simulink model "ECM_1RC_simscape_pulse"  (R2025b)
settings: Solver=ode23t  StartTime=0.0  StopTime=4000  MaxStep=0.1  RelTol=1e-3
libraries: fl_lib x8, nesl_utility x4
settings Model: Creator=klouz  LastModifiedBy=SAT

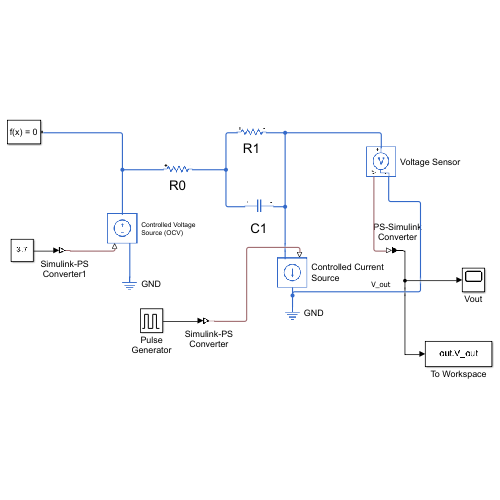
[thumbnail: Simulink's stored preview of the top-level diagram]
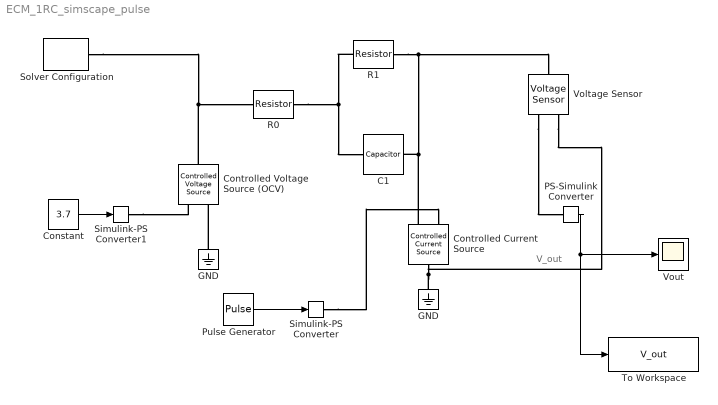
== system ECM_1RC_simscape_pulse ==
  note: V_out
  C1 : fl_lib/Electrical/Electrical Elements/Capacitor  c=1000 F  r=1e-6 Ohm  g=0 1/Ohm  i_specify=off  i_priority=None  i=0 A  i_nominal_specify=off  i_nominal_value=1  i_nominal_unit=A  v_specify=off  v_priority=None  v=0 V  v_nominal_specify=off  v_nominal_value=1  v_nominal_unit=V  vc_specify=off  vc_priority=High  vc=0 V  vc_nominal_specify=off  vc_nominal_value=1  vc_nominal_unit=V
  Constant : Constant  Value=3.7
  Controlled Current Source : fl_lib/Electrical/Electrical Sources/Controlled Current Source
  "Controlled Voltage Source (OCV)  " : fl_lib/Electrical/Electrical Sources/Controlled Voltage Source
  GND : fl_lib/Electrical/Electrical Elements/Electrical Reference
  "GND " : fl_lib/Electrical/Electrical Elements/Electrical Reference
  PS-Simulink Converter : nesl_utility/PS-Simulink Converter  PhysicalDomain=network_engine_domain  SubClassName=ps_output  LeftPortType=input  RightPortType=output  PseudoPeriodic=off  Frequencies=[]  VectorFormat=inherit  Unit=V  AffineConversion=off
  Pulse Generator : DiscretePulseGenerator  PulseType=Time based  Amplitude=5  Period=3000  PulseWidth=3.33  PhaseDelay=600
  R0 : fl_lib/Electrical/Electrical Elements/Resistor  R=0.05 Ohm  i_specify=off  i_priority=None  i=0 A  i_nominal_specify=off  i_nominal_value=1  i_nominal_unit=A  v_specify=off  v_priority=None  v=0 V  v_nominal_specify=off  v_nominal_value=1  v_nominal_unit=V
  R1 : fl_lib/Electrical/Electrical Elements/Resistor  R=0.02 Ohm  i_specify=off  i_priority=None  i=0 A  i_nominal_specify=off  i_nominal_value=1  i_nominal_unit=A  v_specify=off  v_priority=None  v=0 V  v_nominal_specify=off  v_nominal_value=1  v_nominal_unit=V
  Simulink-PS Converter : nesl_utility/Simulink-PS Converter  PhysicalDomain=network_engine_domain  SubClassName=ps_input  LeftPortType=input  RightPortType=output  PseudoPeriodic=off  Frequencies=[]  NoiseDistribution=none  NoiseParameters=[]  Unit=1  AffineConversion=off  FilteringAndDerivatives=provide  SimscapeFilterOrder=1  InputFilterTimeConstant=0.001  UdotUserProvided=0
  Simulink-PS Converter1 : nesl_utility/Simulink-PS Converter  PhysicalDomain=network_engine_domain  SubClassName=ps_input  LeftPortType=input  RightPortType=output  PseudoPeriodic=off  Frequencies=[]  NoiseDistribution=none  NoiseParameters=[]  Unit=1  AffineConversion=off  FilteringAndDerivatives=provide  SimscapeFilterOrder=1  InputFilterTimeConstant=0.001  UdotUserProvided=0
  Solver Configuration : nesl_utility/Solver Configuration  PhysicalDomain=network_engine_domain  SubClassName=solver  LeftPortType=input  RightPortType=generic  Tones=[]  Harmonics=[]  SimulateNoise=off  Profile=off  UseLocalSampling=off  EnableSwitchedLinearOptims=on  FrequencyDomain=off  UseCCode=off  RelTol=0.001  AbsTol=0.001  MinStep=1e-09  ToWorkspace=off  RevertToSquareIcSolve=off  NumHomotopyIterations=100  PhasorMode=off  PhasorModeNumHarmonics=1  ConsistencySolver=NEWTON_XTOL_AFTER_FTOL  IndexReductionMethod=DerivativeReplacement  DoDC=off  ResidualTolerance=1e-09  ConsistencyTolSource=GLOBAL  ConsistencyAbsTol=0.001  ConsistencyRelTol=0.001  ConsistencyTolFactor=0.001  UseLocalSolver=off  LocalSolverChoice=NE_BACKWARD_EULER_ADVANCER  ResolveIndetEquations=on  FunctionEvalNumThread=1  LocalSolverSampleTime=0.001  DoFixedCost=off  MaxNonlinIter=3  MaxModeIter=2  ComputeImpulses=off  ImpulseIterations=2  LinearAlgebra=auto  LinearAlgebraNumThread=0  EquationFormulation=NE_TIME_EF  DelaysMemoryBudget=1024  AutomaticFiltering=on  FilteringTimeConstant=0.001  PartitionStorageMethod=AS_NEEDED  PartitionMemoryBudget=1024  PartitionMethod=ROBUST  MultibodyUseLocalSolver=off  MultibodyLocalSolverChoice=ODE1  MultibodyLocalSolverSampleTime=0.001
  To Workspace : ToWorkspace  VariableName=V_out  SaveFormat=Timeseries  SampleTime=-1
  Voltage Sensor : fl_lib/Electrical/Electrical Sensors/Voltage Sensor
  Vout : Scope
      settings: ActiveDisplayYMinimum=-1  ActiveDisplayYMaximum=1
  wires:
  Pulse Generator/1 -> Simulink-PS Converter/1
  Constant/1 -> Simulink-PS Converter1/1
  PS-Simulink Converter/1 -> To Workspace/1, Vout/1
  connections:
  R1/LConn1 -- R0/RConn1 -- C1/LConn1
  R1/RConn1 -- Voltage Sensor/LConn1 -- Controlled Current Source/RConn2 -- C1/RConn1
  GND/LConn1 -- "Controlled Voltage Source (OCV)  "/RConn2
  "Controlled Voltage Source (OCV)  "/LConn1 -- Solver Configuration/RConn1 -- R0/LConn1
  "GND "/LConn1 -- Voltage Sensor/RConn2 -- Controlled Current Source/LConn1
  Simulink-PS Converter1/RConn1 -- "Controlled Voltage Source (OCV)  "/RConn1
  Simulink-PS Converter/RConn1 -- Controlled Current Source/RConn1
  Voltage Sensor/RConn1 -- PS-Simulink Converter/LConn1
